simulink model "AthletixData_EMG_Simulation"  (R2026b)
settings: Solver=VariableStepAuto  StopTime=5
libraries: simulink x1, cstblocks_varying x1
settings Model: Creator=Maxence  LastModifiedBy=Maxence

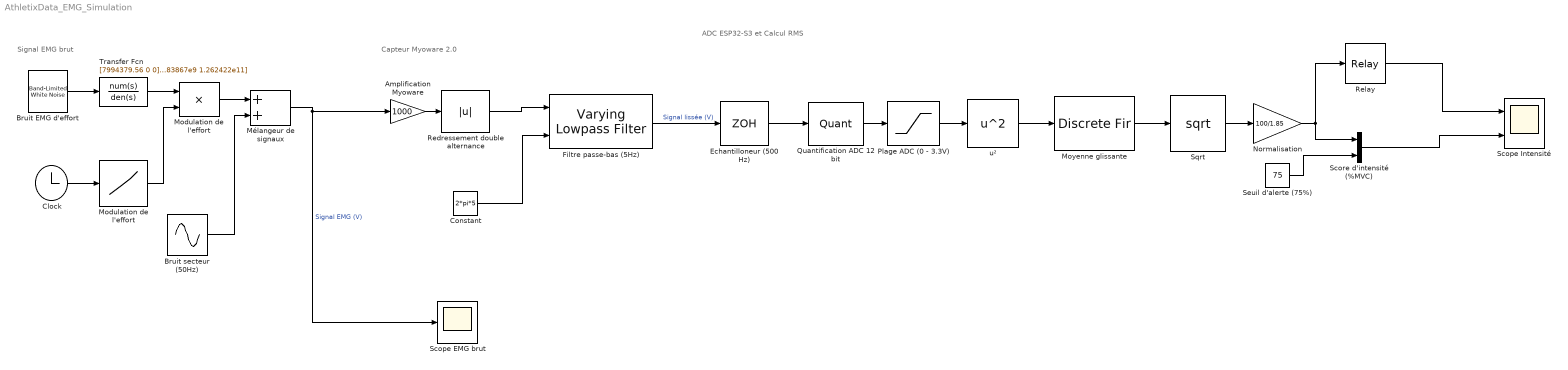
== system AthletixData_EMG_Simulation ==
  note: ADC ESP32-S3 et Calcul RMS
  note: Capteur Myoware 2.0
  note: Signal EMG brut
  Amplification Myoware : Gain  Gain=1000
  Bruit EMG d'effort : simulink/Sources/Band-Limited White Noise  Cov=7.1e-9  Ts=0.0005  seed=[23341]
  Bruit secteur (50Hz) : Sin  Amplitude=0.00008  Frequency=2*pi*50  SampleTime=0
  Clock : Clock
  Constant : Constant  Value=2*pi*5
  Echantilloneur (500 Hz) : ZeroOrderHold  SampleTime=0.002
  Filtre passe-bas (5Hz) : cstblocks_varying/Varying Lowpass Filter  N=2
      settings: LibrarySourceBlock=cstblocks/Linear Parameter Varying/Varying Lowpass Filter
  Modulation de l'effort : Product
  Modulation de l'effort : Lookup_n-D  NumberOfTableDimensions=1  BreakpointsForDimension1=[0 1 1.3 2 2.3 3 3.3 4 4.3 5]  Table=[ 0 0 0.4 0.4 0.95 0.95 0.5 0.5 0 0]  InternalRulePriority=Speed  RndMeth=Simplest
  Moyenne glissante : DiscreteFir  Coefficients=ones(1,100)/100
  "Mélangeur de signaux " : Sum
  Normalisation : Gain  Gain=100/1.85
  Plage ADC (0 - 3.3V) : Saturate  UpperLimit=3.3  LowerLimit=0
  Quantification ADC 12 bit : Quantizer  QuantizationInterval=3.3/4095
  Redressement double alternance : Abs  SaturateOnIntegerOverflow=off
  Relay : Relay  OnSwitchValue=75  OffSwitchValue=70
  Scope EMG brut : Scope
      settings: ActiveDisplayYMinimum=-2.751460957461044  ActiveDisplayYMaximum=2.7748838987048989
  Scope Intensité : Scope  NumInputPorts=2
      settings: ActiveDisplayYMinimum=-0.12499999999999997  ActiveDisplayYMaximum=1.125
  Score d'intensité (%MVC) : Mux  Inputs=2
  "Seuil d'alerte (75%) " : Constant  Value=75
  Sqrt : Sqrt
  Transfer Fcn : TransferFcn  Numerator=[7994379.56 0 0]  Denominator=[1 4176.31 8.720782e6 1.483867e9 1.262422e11]
  u² : Math  Operator=square
  wires:
  Constant/1 -> Filtre passe-bas (5Hz)/2
  Bruit EMG d'effort/1 -> Transfer Fcn/1
  Bruit secteur (50Hz)/1 -> "Mélangeur de signaux "/2
  "Mélangeur de signaux "/1 -> Scope EMG brut/1, Amplification Myoware/1  "Signal EMG (V)"
  Redressement double alternance/1 -> Filtre passe-bas (5Hz)/1
  Filtre passe-bas (5Hz)/1 -> Echantilloneur (500 Hz)/1  "Signal lissée (V)"
  Echantilloneur (500 Hz)/1 -> Quantification ADC 12 bit/1
  Quantification ADC 12 bit/1 -> Plage ADC (0 - 3.3V)/1
  u²/1 -> Moyenne glissante/1
  Moyenne glissante/1 -> Sqrt/1
  Sqrt/1 -> Normalisation/1
  Plage ADC (0 - 3.3V)/1 -> u²/1
  Modulation de l'effort/1 -> "Mélangeur de signaux "/1
  Modulation de l'effort/1 -> Modulation de l'effort/2
  Normalisation/1 -> Relay/1, Score d'intensité (%MVC)/1
  "Seuil d'alerte (75%) "/1 -> Score d'intensité (%MVC)/2
  Relay/1 -> Scope Intensité/1
  Score d'intensité (%MVC)/1 -> Scope Intensité/2
  Transfer Fcn/1 -> Modulation de l'effort/1
  Clock/1 -> Modulation de l'effort/1
  Amplification Myoware/1 -> Redressement double alternance/1
